simulink model "ME486C_Dyno_DAQ_Quality_Development"  (R2025a)
settings: Solver=FixedStepAuto  StartTime=0.0  StopTime=inf  FixedStep=0.02  RelTol=1e-3  EnableMultiTasking=on
libraries: arduinolib x24, simulink x19
(part 1 of 2)
settings Model: SILPILModeSetting=veronly  ExtModeTrigDuration=2  Creator=YHQ  LastModifiedBy=YHQ
settings OptimizationCC: EnhancedBackFolding=on  PassReuseOutputArgsAs=Individual arguments  ZeroExternalMemoryAtStartup=off  ZeroInternalMemoryAtStartup=off  MaxStackSize=64  OptimizeBlockOrder=speed  DifferentSizesBufferReuse=on  OptimizationCustomize=off  EfficientTunableParamExpr=on
settings DebuggingCC: ParameterTunabilityLossMsg=error
settings HardwareCC: ProdBitPerPointer=32.0  ProdBitPerSizeT=32.0  ProdBitPerPtrDiffT=32.0  ProdLargestAtomicInteger=Long  ProdLargestAtomicFloat=Double  ProdWordSize=32.0  ProdLongLongMode=on  ProdHWDeviceType=ARM Compatible->ARM Cortex  UseEmbeddedCoderFeatures=off  UseSimulinkCoderFeatures=off
settings SFSimCC: MATLABDynamicMemAlloc=off
settings RTWCC: SystemTargetFile=ert.tlc  HardwareBoard=Arduino Uno R4 Minima  TemplateMakefile=ert_default_tmf  Toolchain=Arduino ARM M4  BuildConfiguration=Faster Runs  Description=Embedded Coder
settings CodeAppCC: ForceParamTrailComments=on  IgnoreCustomStorageClasses=off  OperatorAnnotations=on  SimulinkDataObjDesc=on  SFDataObjDesc=on  InsertBlockDesc=on
settings ERTTargetCC: ExtModeTransport=3.0  ExtModeAutomaticAllocSize=off  ExtModeStaticAllocSize=8192.0  InlinedParameterPlacement=Hierarchical  SupportContinuousTime=on  SupportNonInlinedSFcns=on  SupportVariableSizeSignals=on

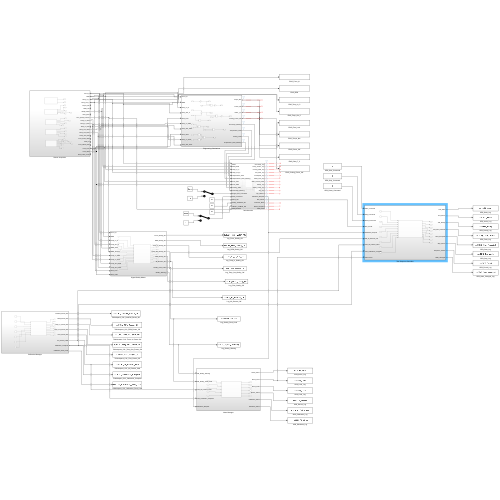
[thumbnail: Simulink's stored preview of the top-level diagram]
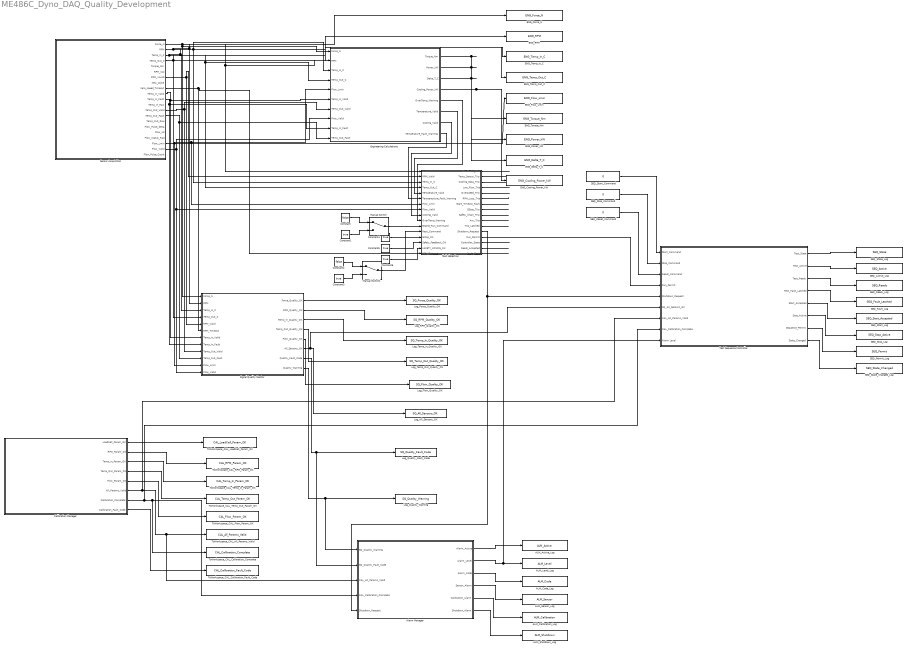
== system ME486C_Dyno_DAQ_Quality_Development ==
  ALM_Active_Log : ToWorkspace  VariableName=ALM_Active  SaveFormat=Timeseries  SampleTime=-1
  ALM_Calibration_Log : ToWorkspace  VariableName=ALM_Calibration  SaveFormat=Timeseries  SampleTime=-1
  ALM_Code_Log : ToWorkspace  VariableName=ALM_Code  SaveFormat=Timeseries  SampleTime=-1
  ALM_Level_Log : ToWorkspace  VariableName=ALM_Level  SaveFormat=Timeseries  SampleTime=-1
  ALM_Sensor_Log : ToWorkspace  VariableName=ALM_Sensor  SaveFormat=Timeseries  SampleTime=-1
  ALM_Shutdown_Log : ToWorkspace  VariableName=ALM_Shutdown  SaveFormat=Timeseries  SampleTime=-1
  Alarm Manager : Subsystem
  Calibration Manager : Subsystem
  Constant : Constant  Value=false  OutDataTypeStr=boolean
  Constant{1,3..6} (5 alike) : Constant  Value=true  OutDataTypeStr=boolean
  Constant2 : Constant  Value=false  OutDataTypeStr=boolean
  ENG_Cooling_Power_kW : ToWorkspace  VariableName=ENG_Cooling_Power_kW  SaveFormat=Timeseries  SampleTime=-1
  ENG_Delta_T_C : ToWorkspace  VariableName=ENG_Delta_T_C  SaveFormat=Timeseries  SampleTime=-1
  ENG_Flow_Lmin : ToWorkspace  VariableName=ENG_Flow_Lmin  SaveFormat=Timeseries  SampleTime=-1
  ENG_Force_N : ToWorkspace  VariableName=ENG_Force_N  SaveFormat=Timeseries  SampleTime=-1
  ENG_Power_kW : ToWorkspace  VariableName=ENG_Power_kW  SaveFormat=Timeseries  SampleTime=-1
  ENG_RPM : ToWorkspace  VariableName=ENG_RPM  SaveFormat=Timeseries  SampleTime=-1
  ENG_Temp_In_C : ToWorkspace  VariableName=ENG_Temp_In_C  SaveFormat=Timeseries  SampleTime=-1
  ENG_Temp_Out_C : ToWorkspace  VariableName=ENG_Temp_Out_C  SaveFormat=Timeseries  SampleTime=-1
  ENG_Torque_Nm : ToWorkspace  VariableName=ENG_Torque_Nm  SaveFormat=Timeseries  SampleTime=-1
  Engineering Calculations : Subsystem
  Log_All_Sensors_OK : ToWorkspace  VariableName=SQ_All_Sensors_OK  SaveFormat=Timeseries  SampleTime=-1
  Log_Flow_Quality_OK : ToWorkspace  VariableName=SQ_Flow_Quality_OK  SaveFormat=Timeseries  SampleTime=-1
  Log_Force_Quality_OK : ToWorkspace  VariableName=SQ_Force_Quality_OK  SaveFormat=Timeseries  SampleTime=-1
  Log_Quality_Fault_Code : ToWorkspace  VariableName=SQ_Quality_Fault_Code  SaveFormat=Timeseries  SampleTime=-1
  Log_Quality_Warning : ToWorkspace  VariableName=SQ_Quality_Warning  SaveFormat=Timeseries  SampleTime=-1
  Log_RPM_Quality_OK : ToWorkspace  VariableName=SQ_RPM_Quality_OK  SaveFormat=Timeseries  SampleTime=-1
  Log_Temp_In_Quality_OK : ToWorkspace  VariableName=SQ_Temp_In_Quality_OK  SaveFormat=Timeseries  SampleTime=-1
  Log_Temp_Out_Quality_OK : ToWorkspace  VariableName=SQ_Temp_Out_Quality_OK  SaveFormat=Timeseries  SampleTime=-1
  Manual Switch : ManualSwitch
  Manual Switch1 : ManualSwitch
  SEQ_Active_Log : ToWorkspace  VariableName=SEQ_Active  SaveFormat=Timeseries  SampleTime=-1
  SEQ_Fault_Log : ToWorkspace  VariableName=SEQ_Fault_Latched  SaveFormat=Timeseries  SampleTime=-1
  SEQ_Permit_Log : ToWorkspace  VariableName=SEQ_Permit  SaveFormat=Timeseries  SampleTime=-1
  SEQ_Ready_Log : ToWorkspace  VariableName=SEQ_Ready  SaveFormat=Timeseries  SampleTime=-1
  SEQ_Reset_Command : Constant  Value=0  OutDataTypeStr=boolean  SampleTime=0.02
  SEQ_Start_Command : Constant  Value=0  OutDataTypeStr=boolean  SampleTime=0.02
  SEQ_Start_Log : ToWorkspace  VariableName=SEQ_Start_Accepted  SaveFormat=Timeseries  SampleTime=-1
  SEQ_State_Changed_Log : ToWorkspace  VariableName=SEQ_State_Changed  SaveFormat=Timeseries  SampleTime=-1
  SEQ_State_Log : ToWorkspace  VariableName=SEQ_State  SaveFormat=Timeseries  SampleTime=-1
  SEQ_Stop_Command : Constant  Value=0  OutDataTypeStr=boolean  SampleTime=0.02
  SEQ_Stop_Log : ToWorkspace  VariableName=SEQ_Stop_Active  SaveFormat=Timeseries  SampleTime=-1
  Sensor Acquisition : Subsystem
  Signal Quality Mentor : Subsystem
  Test Sequence Controller : Subsystem
  ToWorkspace_CAL_All_Params_Valid : ToWorkspace  VariableName=CAL_All_Params_Valid  SaveFormat=Timeseries  SampleTime=-1
  ToWorkspace_CAL_Calibration_Complete : ToWorkspace  VariableName=CAL_Calibration_Complete  SaveFormat=Timeseries  SampleTime=-1
  ToWorkspace_CAL_Calibration_Fault_Code : ToWorkspace  VariableName=CAL_Calibration_Fault_Code  SaveFormat=Timeseries  SampleTime=-1
  ToWorkspace_CAL_Flow_Param_OK : ToWorkspace  VariableName=CAL_Flow_Param_OK  SaveFormat=Timeseries  SampleTime=-1
  ToWorkspace_CAL_LoadCell_Param_OK : ToWorkspace  VariableName=CAL_LoadCell_Param_OK  SaveFormat=Timeseries  SampleTime=-1
  ToWorkspace_CAL_RPM_Param_OK : ToWorkspace  VariableName=CAL_RPM_Param_OK  SaveFormat=Timeseries  SampleTime=-1
  ToWorkspace_CAL_Temp_In_Param_OK : ToWorkspace  VariableName=CAL_Temp_In_Param_OK  SaveFormat=Timeseries  SampleTime=-1
  ToWorkspace_CAL_Temp_Out_Param_OK : ToWorkspace  VariableName=CAL_Temp_Out_Param_OK  SaveFormat=Timeseries  SampleTime=-1
  fault detection : Subsystem
  wires:
  Sensor Acquisition/1(Force_N) -> Engineering Calculations/1(Force_N), Signal Quality Mentor/1(Force_N), ENG_Force_N/1
  Sensor Acquisition/2(RPM) -> fault detection/1(RPM), Engineering Calculations/2(RPM), Signal Quality Mentor/2(RPM), ENG_RPM/1
  Sensor Acquisition/3(Temp_In_C) -> fault detection/3(Temp_In_C), Engineering Calculations/3(Temp_In_C), Signal Quality Mentor/3(Temp_In_C), ENG_Temp_In_C/1
  Sensor Acquisition/4(Temp_Out_C) -> ENG_Temp_Out_C/1, fault detection/4(Temp_Out_C), Engineering Calculations/4(Temp_Out_C), Signal Quality Mentor/4(Temp_Out_C)
  Sensor Acquisition/19(Flow_Lmin) -> ENG_Flow_Lmin/1, Engineering Calculations/5(Flow_Lmin), fault detection/7(Flow_Lmin), Signal Quality Mentor/11(Flow_Lmin)
  Sensor Acquisition/10(Temp_In_Valid) -> Engineering Calculations/6(Temp_In_Valid), Signal Quality Mentor/7(Temp_In_Valid)
  Sensor Acquisition/13(Temp_Out_Valid) -> Engineering Calculations/7(Temp_Out_Valid), Signal Quality Mentor/9(Temp_Out_Valid)
  Sensor Acquisition/11(Temp_In_Fault) -> Engineering Calculations/9(Temp_In_Fault), Signal Quality Mentor/8(Temp_In_Fault)
  Sensor Acquisition/14(Temp_Out_Fault) -> Engineering Calculations/10(Temp_Out_Fault), Signal Quality Mentor/10(Temp_Out_Fault)
  Engineering Calculations/6(Temperature_Valid) -> fault detection/5(Temperature_Valid)
  Engineering Calculations/7(Cooling_Valid) -> fault detection/9(Cooling_Valid)
  Engineering Calculations/8(Temperature_Fault_Warning) -> fault detection/6(Temperasture_Fault_Warning)
  Sensor Acquisition/7(RPM_VALID) -> fault detection/2(RPM_Valid), Signal Quality Mentor/5(RPM_Valid)
  Sensor Acquisition/9(zero_speed_Timeout) -> Signal Quality Mentor/6(RPM_Timeout), fault detection/16(RPM_Timeout)
  Constant/1 -> Manual Switch/1
  Constant1/1 -> Manual Switch/2
  Manual Switch/1 -> fault detection/11(Engine_Run_Command)
  Constant3/1 -> Manual Switch1/2
  Constant2/1 -> Manual Switch1/1
  Manual Switch1/1 -> fault detection/12(Rest_Command)
  Constant4/1 -> fault detection/13(Estop_OK)
  Constant5/1 -> fault detection/14(Safety_Feedback_OK)
  Constant6/1 -> fault detection/15(sAFETY_cONFIG_OK)
  Engineering Calculations/5(OverTemp_Warning) -> fault detection/10(OverTemp_Warning)
  fault detection/1(OverTemp_Trip) -> ?
  fault detection/2(Temp_Sensor_Trip) -> ?
  fault detection/3(Cooling_Data_Trip) -> ?
  fault detection/4(Low_Flow_Trip) -> ?
  fault detection/5(Overspeed_Trip) -> ?
  fault detection/6(RPM_Loss_Trip) -> ?
  fault detection/7(Start_Timeout_Fault) -> ?
  fault detection/8(EStop_Trip) -> ?
  fault detection/9(Safety_Chain_Trip) -> ?
  fault detection/10(Any_Trip) -> ?
  fault detection/11(Trip_Latched) -> ?
  fault detection/12(Shutdown_Request) -> Alarm Manager/5(Shutdown_Request), Test Sequence Controller/5(Shutdown_Request)
  fault detection/13(Run_Permit) -> Test Sequence Controller/4(Run_Permit)
  fault detection/14(Controller_State) -> ?
  fault detection/15(Reset_Accepted) -> ?
  fault detection/16(Fault_Code) -> ?
  Engineering Calculations/1(Torque_Nm) -> ENG_Torque_Nm/1
  Engineering Calculations/2(Power_kW) -> ENG_Power_kW/1
  Engineering Calculations/3(Delta_T_C) -> ENG_Delta_T_C/1
  Engineering Calculations/4(Cooling_Power_kW) -> ENG_Cooling_Power_kW/1
  Sensor Acquisition/20(Flow_Valid) -> Engineering Calculations/8(Flow_Valid), Signal Quality Mentor/12(Flow_Valid), fault detection/8(Flow_Valid)
  Signal Quality Mentor/1(Force_Quality_OK) -> Log_Force_Quality_OK/1
  Signal Quality Mentor/2(RPM_Quality_OK) -> Log_RPM_Quality_OK/1
  Signal Quality Mentor/3(Temp_In_Quality_OK) -> Log_Temp_In_Quality_OK/1
  Signal Quality Mentor/4(Temp_Out_Quality_OK) -> Log_Temp_Out_Quality_OK/1
  Signal Quality Mentor/5(Flow_Quality_OK) -> Log_Flow_Quality_OK/1
  Signal Quality Mentor/6(All_Sensors_OK) -> Test Sequence Controller/6(SQ_All_Sensors_OK), Log_All_Sensors_OK/1
  Signal Quality Mentor/7(Quality_Fault_Code) -> Alarm Manager/2(SQ_Quality_Fault_Code), Log_Quality_Fault_Code/1
  Signal Quality Mentor/8(Quality_Warning) -> Alarm Manager/1(SQ_Quality_Warning), Log_Quality_Warning/1
  Calibration Manager/1(LoadCell_Param_OK) -> ToWorkspace_CAL_LoadCell_Param_OK/1
  Calibration Manager/2(RPM_Param_OK) -> ToWorkspace_CAL_RPM_Param_OK/1
  Calibration Manager/3(Temp_In_Param_OK) -> ToWorkspace_CAL_Temp_In_Param_OK/1
  Calibration Manager/4(Temp_Out_Param_OK) -> ToWorkspace_CAL_Temp_Out_Param_OK/1
  Calibration Manager/5(Flow_Param_OK) -> ToWorkspace_CAL_Flow_Param_OK/1
  Calibration Manager/6(All_Params_Valid) -> Test Sequence Controller/7(CAL_All_Params_Valid), Alarm Manager/3(CAL_All_Params_Valid), ToWorkspace_CAL_All_Params_Valid/1
  Calibration Manager/7(Calibration_Complete) -> Alarm Manager/4(CAL_Calibration_Complete), ToWorkspace_CAL_Calibration_Complete/1, Test Sequence Controller/8(CAL_Calibration_Complete)
  Calibration Manager/8(Calibration_Fault_Code) -> ToWorkspace_CAL_Calibration_Fault_Code/1
  Alarm Manager/1(Alarm_Active) -> ALM_Active_Log/1
  Alarm Manager/2(Alarm_Level) -> Test Sequence Controller/9(Alarm Level), ALM_Level_Log/1
  Alarm Manager/3(Alarm_Code) -> ALM_Code_Log/1
  Alarm Manager/4(Sensor_Alarm) -> ALM_Sensor_Log/1
  Alarm Manager/5(Calibration_Alarm) -> ALM_Calibration_Log/1
  Alarm Manager/6(Shutdown_Alarm) -> ALM_Shutdown_Log/1
  SEQ_Start_Command/1 -> Test Sequence Controller/1(Start_Command)
  SEQ_Stop_Command/1 -> Test Sequence Controller/2(Stop_Command)
  SEQ_Reset_Command/1 -> Test Sequence Controller/3(Reset_Command)
  Test Sequence Controller/1(Test_State) -> SEQ_State_Log/1
  Test Sequence Controller/2(Test_Active) -> SEQ_Active_Log/1
  Test Sequence Controller/3(Test_Ready) -> SEQ_Ready_Log/1
  Test Sequence Controller/4(Test_Fault_Latched) -> SEQ_Fault_Log/1
  Test Sequence Controller/5(Start_Accepted) -> SEQ_Start_Log/1
  Test Sequence Controller/6(Stop_Active) -> SEQ_Stop_Log/1
  Test Sequence Controller/7(Sequence_Permit) -> SEQ_Permit_Log/1
  Test Sequence Controller/8(State_Changed) -> SEQ_State_Changed_Log/1

== system ME486C_Dyno_DAQ_Quality_Development/Alarm Manager ==
  SQ_Quality_Warning : Inport
  SQ_Quality_Fault_Code : Inport  Port=2
  CAL_All_Params_Valid : Inport  Port=3
  CAL_Calibration_Complete : Inport  Port=4
  Shutdown_Request : Inport  Port=5
  Alarm_Logic_Core : MATLAB Function  TreatAsAtomicUnit=on
  Alarm_Active : Outport
  Alarm_Level : Outport  Port=2
  Alarm_Code : Outport  Port=3
  Sensor_Alarm : Outport  Port=4
  Calibration_Alarm : Outport  Port=5
  Shutdown_Alarm : Outport  Port=6
  wires:
  Shutdown_Request/1 -> Alarm_Logic_Core/5(Shutdown_Request)
  CAL_Calibration_Complete/1 -> Alarm_Logic_Core/4(CAL_Calibration_Complete)
  CAL_All_Params_Valid/1 -> Alarm_Logic_Core/3(CAL_All_Params_Valid)
  SQ_Quality_Fault_Code/1 -> Alarm_Logic_Core/2(SQ_Quality_Fault_Code)
  SQ_Quality_Warning/1 -> Alarm_Logic_Core/1(SQ_Quality_Warning)
  Alarm_Logic_Core/1(Alarm_Active) -> Alarm_Active/1
  Alarm_Logic_Core/2(Alarm_Level) -> Alarm_Level/1
  Alarm_Logic_Core/3(Alarm_Code) -> Alarm_Code/1
  Alarm_Logic_Core/4(Sensor_Alarm) -> Sensor_Alarm/1
  Alarm_Logic_Core/5(Calibration_Alarm) -> Calibration_Alarm/1
  Alarm_Logic_Core/6(Shutdown_Alarm) -> Shutdown_Alarm/1

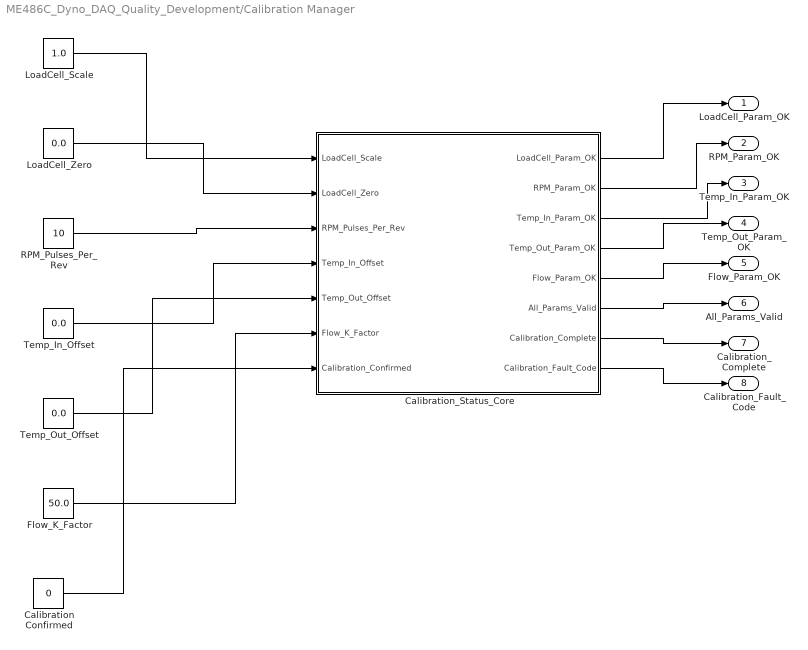
== system ME486C_Dyno_DAQ_Quality_Development/Calibration Manager ==
  Calibration Confirmed : Constant  Value=0  OutDataTypeStr=boolean
  Calibration_Status_Core : MATLAB Function  TreatAsAtomicUnit=on
  Flow_K_Factor : Constant  Value=50.0
  LoadCell_Scale : Constant  Value=1.0
  LoadCell_Zero : Constant  Value=0.0
  RPM_Pulses_Per_Rev : Constant  Value=10
  Temp_In_Offset : Constant  Value=0.0
  Temp_Out_Offset : Constant  Value=0.0
  LoadCell_Param_OK : Outport
  RPM_Param_OK : Outport  Port=2
  Temp_In_Param_OK : Outport  Port=3
  Temp_Out_Param_OK : Outport  Port=4
  Flow_Param_OK : Outport  Port=5
  All_Params_Valid : Outport  Port=6
  Calibration_Complete : Outport  Port=7
  Calibration_Fault_Code : Outport  Port=8
  wires:
  LoadCell_Scale/1 -> Calibration_Status_Core/1(LoadCell_Scale)
  LoadCell_Zero/1 -> Calibration_Status_Core/2(LoadCell_Zero)
  RPM_Pulses_Per_Rev/1 -> Calibration_Status_Core/3(RPM_Pulses_Per_Rev)
  Temp_In_Offset/1 -> Calibration_Status_Core/4(Temp_In_Offset)
  Temp_Out_Offset/1 -> Calibration_Status_Core/5(Temp_Out_Offset)
  Flow_K_Factor/1 -> Calibration_Status_Core/6(Flow_K_Factor)
  Calibration_Status_Core/1(LoadCell_Param_OK) -> LoadCell_Param_OK/1
  Calibration_Status_Core/2(RPM_Param_OK) -> RPM_Param_OK/1
  Calibration_Status_Core/3(Temp_In_Param_OK) -> Temp_In_Param_OK/1
  Calibration_Status_Core/4(Temp_Out_Param_OK) -> Temp_Out_Param_OK/1
  Calibration_Status_Core/5(Flow_Param_OK) -> Flow_Param_OK/1
  Calibration_Status_Core/6(All_Params_Valid) -> All_Params_Valid/1
  Calibration_Status_Core/7(Calibration_Complete) -> Calibration_Complete/1
  Calibration_Status_Core/8(Calibration_Fault_Code) -> Calibration_Fault_Code/1
  Calibration Confirmed/1 -> Calibration_Status_Core/7(Calibration_Confirmed)

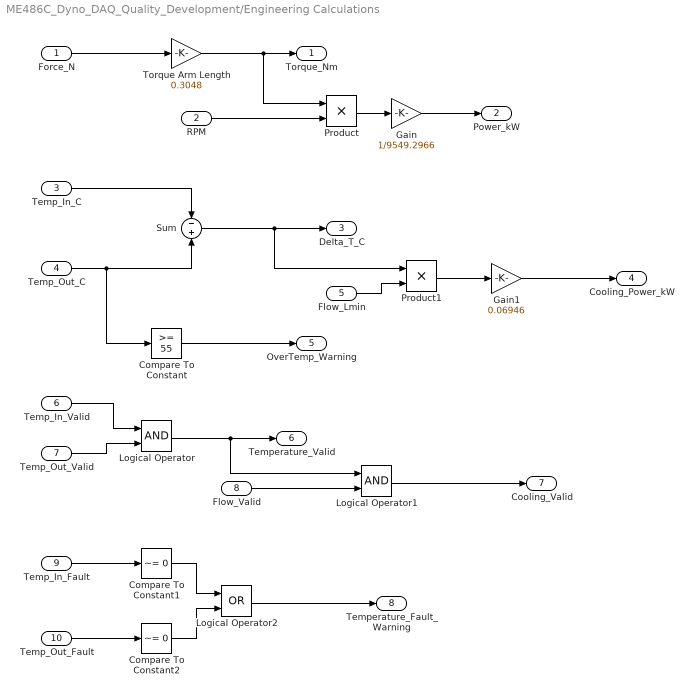
== system ME486C_Dyno_DAQ_Quality_Development/Engineering Calculations ==
  Force_N : Inport
  RPM : Inport  Port=2
  Temp_In_C : Inport  Port=3
  Temp_Out_C : Inport  Port=4
  Flow_Lmin : Inport  Port=5
  Temp_In_Valid : Inport  Port=6
  Temp_Out_Valid : Inport  Port=7
  Flow_Valid : Inport  Port=8
  Temp_In_Fault : Inport  Port=9
  Temp_Out_Fault : Inport  Port=10
  Compare To Constant : simulink/Logic and Bit Operations/Compare To Constant  relop=>=  const=55  OutDataTypeStr=boolean
  Compare To Constant1 : simulink/Logic and Bit Operations/Compare To Constant  relop=~=  const=0  OutDataTypeStr=boolean
  Compare To Constant2 : simulink/Logic and Bit Operations/Compare To Constant  relop=~=  const=0  OutDataTypeStr=boolean
  Gain : Gain  Gain=1/9549.2966
  Gain1 : Gain  Gain=0.06946
  Logical Operator : Logic  AllPortsSameDT=off  OutDataTypeStr=boolean
  Logical Operator1 : Logic  AllPortsSameDT=off  OutDataTypeStr=boolean
  Logical Operator2 : Logic  Operator=OR  AllPortsSameDT=off  OutDataTypeStr=boolean
  Product : Product
  Product1 : Product
  Sum : Sum  Inputs=-+
  Torque Arm Length : Gain  Gain=0.3048
  Torque_Nm : Outport
  Power_kW : Outport  Port=2
  Delta_T_C : Outport  Port=3
  Cooling_Power_kW : Outport  Port=4
  OverTemp_Warning : Outport  Port=5
  Temperature_Valid : Outport  Port=6
  Cooling_Valid : Outport  Port=7
  Temperature_Fault_Warning : Outport  Port=8
  wires:
  Force_N/1 -> Torque Arm Length/1
  Torque Arm Length/1 -> Product/1, Torque_Nm/1
  RPM/1 -> Product/2
  Product/1 -> Gain/1
  Gain/1 -> Power_kW/1
  Temp_In_C/1 -> Sum/1
  Temp_Out_C/1 -> Compare To Constant/1, Sum/2
  Sum/1 -> Product1/1, Delta_T_C/1
  Flow_Lmin/1 -> Product1/2
  Product1/1 -> Gain1/1
  Gain1/1 -> Cooling_Power_kW/1
  Compare To Constant/1 -> OverTemp_Warning/1
  Temp_In_Valid/1 -> Logical Operator/1
  Temp_Out_Valid/1 -> Logical Operator/2
  Logical Operator/1 -> Logical Operator1/1, Temperature_Valid/1
  Flow_Valid/1 -> Logical Operator1/2
  Logical Operator1/1 -> Cooling_Valid/1
  Temp_In_Fault/1 -> Compare To Constant1/1
  Temp_Out_Fault/1 -> Compare To Constant2/1
  Compare To Constant1/1 -> Logical Operator2/1
  Compare To Constant2/1 -> Logical Operator2/2
  Logical Operator2/1 -> Temperature_Fault_Warning/1

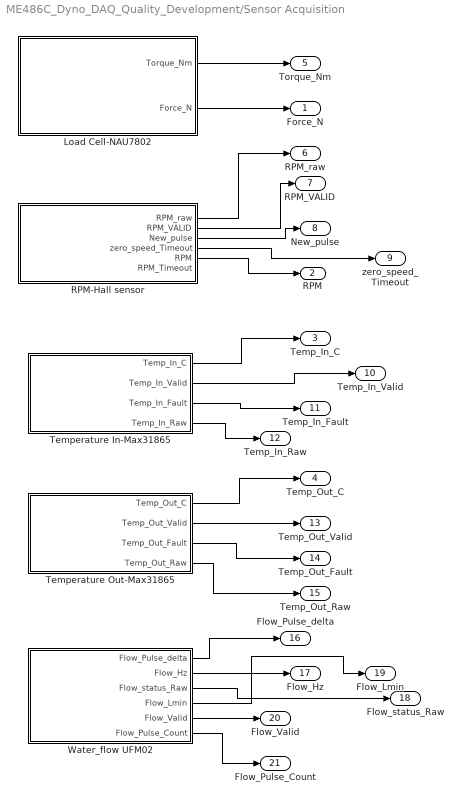
== system ME486C_Dyno_DAQ_Quality_Development/Sensor Acquisition ==
  Load Cell-NAU7802 : Subsystem
  RPM-Hall sensor : Subsystem
  Temperature In-Max31865 : Subsystem
  Temperature Out-Max31865 : Subsystem
  Water_flow UFM02 : Subsystem
  Force_N : Outport
  RPM : Outport  Port=2
  Temp_In_C : Outport  Port=3
  Temp_Out_C : Outport  Port=4
  Torque_Nm : Outport  Port=5
  RPM_raw : Outport  Port=6
  RPM_VALID : Outport  Port=7
  New_pulse : Outport  Port=8
  zero_speed_Timeout : Outport  Port=9
  Temp_In_Valid : Outport  Port=10
  Temp_In_Fault : Outport  Port=11
  Temp_In_Raw : Outport  Port=12
  Temp_Out_Valid : Outport  Port=13
  Temp_Out_Fault : Outport  Port=14
  Temp_Out_Raw : Outport  Port=15
  Flow_Pulse_delta : Outport  Port=16
  Flow_Hz : Outport  Port=17
  Flow_status_Raw : Outport  Port=18
  Flow_Lmin : Outport  Port=19
  Flow_Valid : Outport  Port=20
  Flow_Pulse_Count : Outport  Port=21
  wires:
  Load Cell-NAU7802/2(Force_N) -> Force_N/1
  RPM-Hall sensor/5(RPM) -> RPM/1
  Temperature In-Max31865/1(Temp_In_C) -> Temp_In_C/1
  Temperature Out-Max31865/1(Temp_Out_C) -> Temp_Out_C/1
  Load Cell-NAU7802/1(Torque_Nm) -> Torque_Nm/1
  RPM-Hall sensor/1(RPM_raw) -> RPM_raw/1
  RPM-Hall sensor/2(RPM_VALID) -> RPM_VALID/1
  RPM-Hall sensor/3(New_pulse) -> New_pulse/1
  RPM-Hall sensor/4(zero_speed_Timeout) -> zero_speed_Timeout/1
  Temperature In-Max31865/2(Temp_In_Valid) -> Temp_In_Valid/1
  Temperature In-Max31865/3(Temp_In_Fault) -> Temp_In_Fault/1
  Temperature In-Max31865/4(Temp_In_Raw) -> Temp_In_Raw/1
  Temperature Out-Max31865/2(Temp_Out_Valid) -> Temp_Out_Valid/1
  Temperature Out-Max31865/3(Temp_Out_Fault) -> Temp_Out_Fault/1
  Temperature Out-Max31865/4(Temp_Out_Raw) -> Temp_Out_Raw/1
  Water_flow UFM02/1(Flow_Pulse_delta) -> Flow_Pulse_delta/1
  Water_flow UFM02/2(Flow_Hz) -> Flow_Hz/1
  Water_flow UFM02/3(Flow_status_Raw) -> Flow_status_Raw/1
  Water_flow UFM02/4(Flow_Lmin) -> Flow_Lmin/1
  Water_flow UFM02/5(Flow_Valid) -> Flow_Valid/1
  Water_flow UFM02/6(Flow_Pulse_Count) -> Flow_Pulse_Count/1

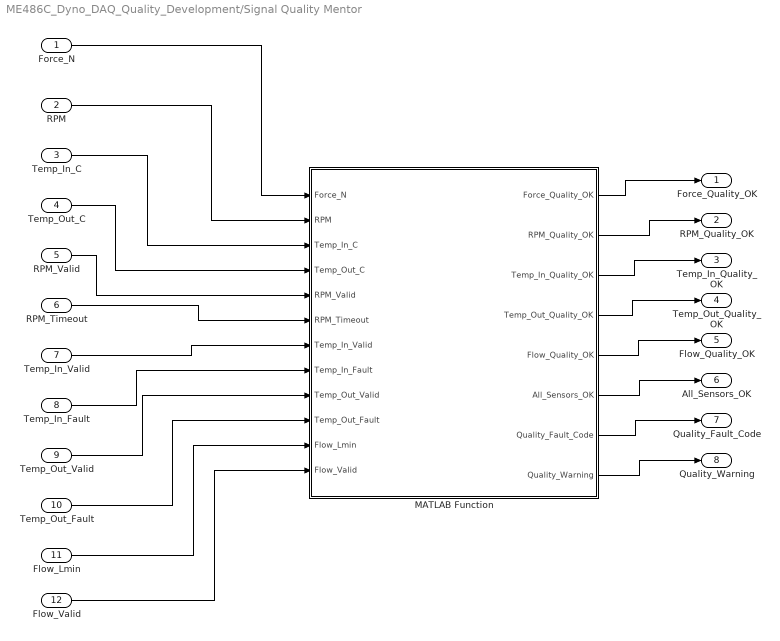
== system ME486C_Dyno_DAQ_Quality_Development/Signal Quality Mentor ==
  Force_N : Inport
  RPM : Inport  Port=2
  Temp_In_C : Inport  Port=3
  Temp_Out_C : Inport  Port=4
  RPM_Valid : Inport  Port=5
  RPM_Timeout : Inport  Port=6
  Temp_In_Valid : Inport  Port=7
  Temp_In_Fault : Inport  Port=8
  Temp_Out_Valid : Inport  Port=9
  Temp_Out_Fault : Inport  Port=10
  Flow_Lmin : Inport  Port=11
  Flow_Valid : Inport  Port=12
  MATLAB Function : MATLAB Function  TreatAsAtomicUnit=on
  Force_Quality_OK : Outport
  RPM_Quality_OK : Outport  Port=2
  Temp_In_Quality_OK : Outport  Port=3
  Temp_Out_Quality_OK : Outport  Port=4
  Flow_Quality_OK : Outport  Port=5
  All_Sensors_OK : Outport  Port=6
  Quality_Fault_Code : Outport  Port=7
  Quality_Warning : Outport  Port=8
  wires:
  Force_N/1 -> MATLAB Function/1(Force_N)
  RPM/1 -> MATLAB Function/2(RPM)
  MATLAB Function/1(Force_Quality_OK) -> Force_Quality_OK/1
  MATLAB Function/2(RPM_Quality_OK) -> RPM_Quality_OK/1
  Temp_In_C/1 -> MATLAB Function/3(Temp_In_C)
  Temp_Out_C/1 -> MATLAB Function/4(Temp_Out_C)
  RPM_Valid/1 -> MATLAB Function/5(RPM_Valid)
  RPM_Timeout/1 -> MATLAB Function/6(RPM_Timeout)
  Temp_In_Valid/1 -> MATLAB Function/7(Temp_In_Valid)
  Temp_In_Fault/1 -> MATLAB Function/8(Temp_In_Fault)
  Temp_Out_Valid/1 -> MATLAB Function/9(Temp_Out_Valid)
  Temp_Out_Fault/1 -> MATLAB Function/10(Temp_Out_Fault)
  Flow_Lmin/1 -> MATLAB Function/11(Flow_Lmin)
  Flow_Valid/1 -> MATLAB Function/12(Flow_Valid)
  MATLAB Function/3(Temp_In_Quality_OK) -> Temp_In_Quality_OK/1
  MATLAB Function/4(Temp_Out_Quality_OK) -> Temp_Out_Quality_OK/1
  MATLAB Function/5(Flow_Quality_OK) -> Flow_Quality_OK/1
  MATLAB Function/6(All_Sensors_OK) -> All_Sensors_OK/1
  MATLAB Function/7(Quality_Fault_Code) -> Quality_Fault_Code/1
  MATLAB Function/8(Quality_Warning) -> Quality_Warning/1

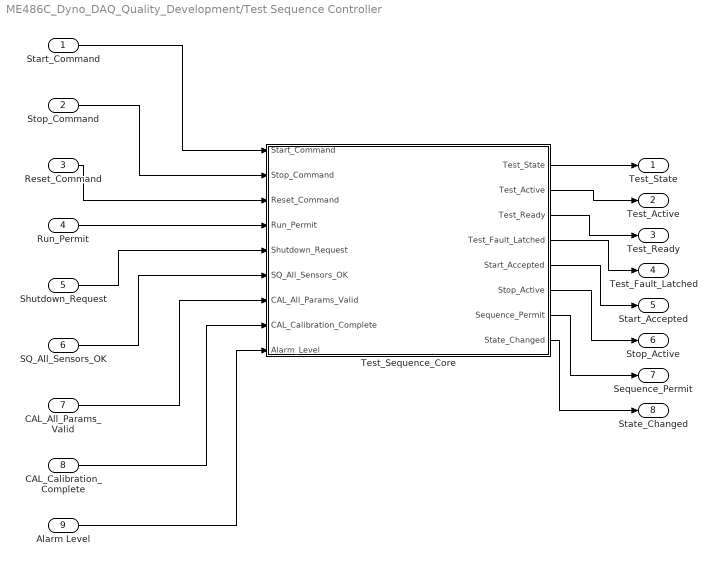
== system ME486C_Dyno_DAQ_Quality_Development/Test Sequence Controller ==
  Start_Command : Inport
  Stop_Command : Inport  Port=2
  Reset_Command : Inport  Port=3
  Run_Permit : Inport  Port=4
  Shutdown_Request : Inport  Port=5
  SQ_All_Sensors_OK : Inport  Port=6
  CAL_All_Params_Valid : Inport  Port=7
  CAL_Calibration_Complete : Inport  Port=8
  Alarm Level : Inport  Port=9
  Test_Sequence_Core : MATLAB Function  TreatAsAtomicUnit=on
  Test_State : Outport
  Test_Active : Outport  Port=2
  Test_Ready : Outport  Port=3
  Test_Fault_Latched : Outport  Port=4
  Start_Accepted : Outport  Port=5
  Stop_Active : Outport  Port=6
  Sequence_Permit : Outport  Port=7
  State_Changed : Outport  Port=8
  wires:
  Start_Command/1 -> Test_Sequence_Core/1(Start_Command)
  Stop_Command/1 -> Test_Sequence_Core/2(Stop_Command)
  Reset_Command/1 -> Test_Sequence_Core/3(Reset_Command)
  Run_Permit/1 -> Test_Sequence_Core/4(Run_Permit)
  Shutdown_Request/1 -> Test_Sequence_Core/5(Shutdown_Request)
  SQ_All_Sensors_OK/1 -> Test_Sequence_Core/6(SQ_All_Sensors_OK)
  CAL_All_Params_Valid/1 -> Test_Sequence_Core/7(CAL_All_Params_Valid)
  CAL_Calibration_Complete/1 -> Test_Sequence_Core/8(CAL_Calibration_Complete)
  Alarm Level/1 -> Test_Sequence_Core/9(Alarm_Level)
  Test_Sequence_Core/1(Test_State) -> Test_State/1
  Test_Sequence_Core/2(Test_Active) -> Test_Active/1
  Test_Sequence_Core/3(Test_Ready) -> Test_Ready/1
  Test_Sequence_Core/4(Test_Fault_Latched) -> Test_Fault_Latched/1
  Test_Sequence_Core/5(Start_Accepted) -> Start_Accepted/1
  Test_Sequence_Core/6(Stop_Active) -> Stop_Active/1
  Test_Sequence_Core/7(Sequence_Permit) -> Sequence_Permit/1
  Test_Sequence_Core/8(State_Changed) -> State_Changed/1

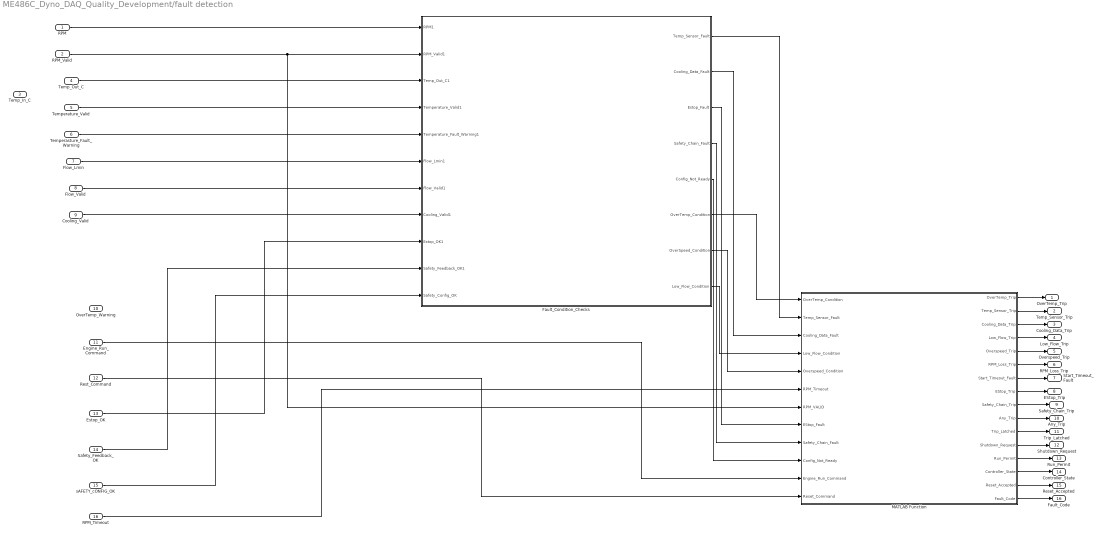
== system ME486C_Dyno_DAQ_Quality_Development/fault detection ==
  RPM : Inport
  RPM_Valid : Inport  Port=2
  Temp_In_C : Inport  Port=3
  Temp_Out_C : Inport  Port=4
  Temperature_Valid : Inport  Port=5
  Temperasture_Fault_Warning : Inport  Port=6
  Flow_Lmin : Inport  Port=7
  Flow_Valid : Inport  Port=8
  Cooling_Valid : Inport  Port=9
  OverTemp_Warning : Inport  Port=10
  Engine_Run_Command : Inport  Port=11
  Rest_Command : Inport  Port=12
  Estop_OK : Inport  Port=13
  Safety_Feedback_OK : Inport  Port=14
  sAFETY_cONFIG_OK : Inport  Port=15
  RPM_Timeout : Inport  Port=16
  Fault_Condition_Checks : Subsystem
  MATLAB Function : MATLAB Function  TreatAsAtomicUnit=on
  OverTemp_Trip : Outport
  Temp_Sensor_Trip : Outport  Port=2
  Cooling_Data_Trip : Outport  Port=3
  Low_Flow_Trip : Outport  Port=4
  Overspeed_Trip : Outport  Port=5
  RPM_Loss_Trip : Outport  Port=6
  Start_Timeout_Fault : Outport  Port=7
  EStop_Trip : Outport  Port=8
  Safety_Chain_Trip : Outport  Port=9
  Any_Trip : Outport  Port=10
  Trip_Latched : Outport  Port=11
  Shutdown_Request : Outport  Port=12
  Run_Permit : Outport  Port=13
  Controller_State : Outport  Port=14
  Reset_Accepted : Outport  Port=15
  Fault_Code : Outport  Port=16
  wires:
  RPM/1 -> Fault_Condition_Checks/1(RPM1)
  RPM_Valid/1 -> MATLAB Function/7(RPM_VALID), Fault_Condition_Checks/2(RPM_Valid1)
  Temp_Out_C/1 -> Fault_Condition_Checks/3(Temp_Out_C1)
  Temperature_Valid/1 -> Fault_Condition_Checks/4(Temperature_Valid1)
  Temperasture_Fault_Warning/1 -> Fault_Condition_Checks/5(Temperature_Fault_Warning1)
  Flow_Lmin/1 -> Fault_Condition_Checks/6(Flow_Lmin1)
  Flow_Valid/1 -> Fault_Condition_Checks/7(Flow_Valid1)
  Cooling_Valid/1 -> Fault_Condition_Checks/8(Cooling_Valid1)
  Estop_OK/1 -> Fault_Condition_Checks/9(Estop_OK1)
  Safety_Feedback_OK/1 -> Fault_Condition_Checks/10(Safety_Feedback_OK1)
  sAFETY_cONFIG_OK/1 -> Fault_Condition_Checks/11(Safety_Config_OK)
  RPM_Timeout/1 -> MATLAB Function/6(RPM_Timeout)
  Engine_Run_Command/1 -> MATLAB Function/11(Engine_Run_Command)
  Rest_Command/1 -> MATLAB Function/12(Reset_Command)
  Fault_Condition_Checks/6(OverTemp_Condition) -> MATLAB Function/1(OverTemp_Condition)
  Fault_Condition_Checks/1(Temp_Sensor_Fault) -> MATLAB Function/2(Temp_Sensor_Fault)
  Fault_Condition_Checks/2(Cooling_Data_Fault) -> MATLAB Function/3(Cooling_Data_Fault)
  Fault_Condition_Checks/3(Estop_Fault) -> MATLAB Function/8(EStop_Fault)
  Fault_Condition_Checks/4(Safety_Chain_Fault) -> MATLAB Function/9(Safety_Chain_Fault)
  Fault_Condition_Checks/5(Config_Not_Ready) -> MATLAB Function/10(Config_Not_Ready)
  Fault_Condition_Checks/8(Low_Flow_Condition) -> MATLAB Function/4(Low_Flow_Condition)
  Fault_Condition_Checks/7(OverSpeed_Condition) -> MATLAB Function/5(Overspeed_Condition)
  MATLAB Function/1(OverTemp_Trip) -> OverTemp_Trip/1
  MATLAB Function/2(Temp_Sensor_Trip) -> Temp_Sensor_Trip/1
  MATLAB Function/3(Cooling_Data_Trip) -> Cooling_Data_Trip/1
  MATLAB Function/4(Low_Flow_Trip) -> Low_Flow_Trip/1
  MATLAB Function/5(Overspeed_Trip) -> Overspeed_Trip/1
  MATLAB Function/6(RPM_Loss_Trip) -> RPM_Loss_Trip/1
  MATLAB Function/7(Start_Timeout_Fault) -> Start_Timeout_Fault/1
  MATLAB Function/8(EStop_Trip) -> EStop_Trip/1
  MATLAB Function/9(Safety_Chain_Trip) -> Safety_Chain_Trip/1
  MATLAB Function/10(Any_Trip) -> Any_Trip/1
  MATLAB Function/11(Trip_Latched) -> Trip_Latched/1
  MATLAB Function/12(Shutdown_Request) -> Shutdown_Request/1
  MATLAB Function/13(Run_Permit) -> Run_Permit/1
  MATLAB Function/14(Controller_State) -> Controller_State/1
  MATLAB Function/15(Reset_Accepted) -> Reset_Accepted/1
  MATLAB Function/16(Fault_Code) -> Fault_Code/1

== system ME486C_Dyno_DAQ_Quality_Development/Sensor Acquisition/Load Cell-NAU7802 ==
  ADC Data read : Subsystem  TreatAsAtomicUnit=on
  Logical Operator : Logic  AllPortsSameDT=off  OutDataTypeStr=boolean
  NAU7802 Initialization : Subsystem
  Torque Arm length : Gain  Gain=0.3048
  Torque_Nm : Outport
  Force_N : Outport  Port=2
  wires:
  NAU7802 Initialization/2(CR_Status) -> Logical Operator/1
  NAU7802 Initialization/6(Calibration done) -> Logical Operator/2
  Logical Operator/1 -> ADC Data read/Enable
  Torque Arm length/1 -> Torque_Nm/1
  ADC Data read/5(Force_N) -> Force_N/1, Torque Arm length/1

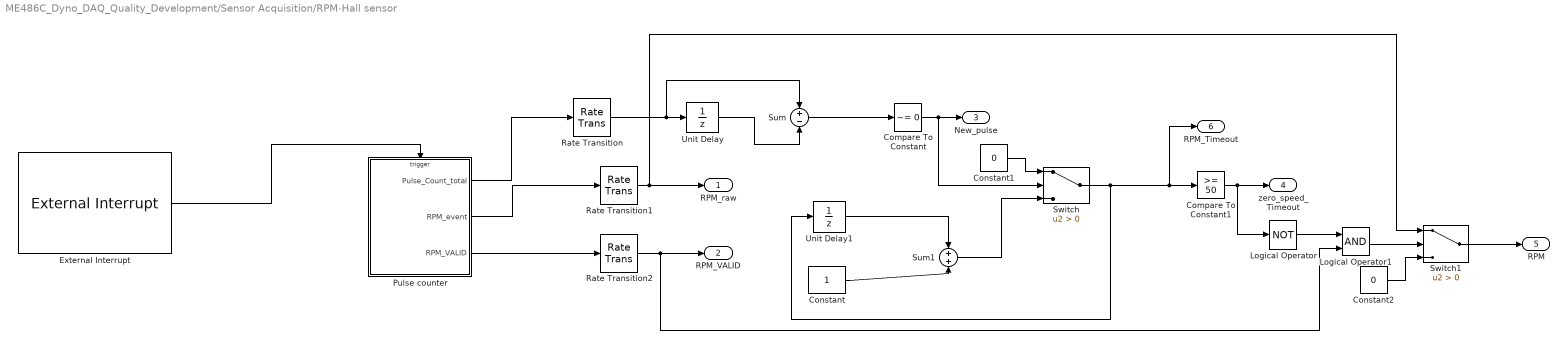
== system ME486C_Dyno_DAQ_Quality_Development/Sensor Acquisition/RPM-Hall sensor ==
  Compare To Constant : simulink/Logic and Bit Operations/Compare To Constant  relop=~=  const=0  OutDataTypeStr=boolean
  Compare To Constant1 : simulink/Logic and Bit Operations/Compare To Constant  relop=>=  const=50  OutDataTypeStr=boolean
  Constant : Constant  OutDataTypeStr=uint16
  Constant1 : Constant  Value=0  OutDataTypeStr=uint16
  Constant2 : Constant  Value=0  OutDataTypeStr=uint16
  External Interrupt : arduinolib/External Interrupt  Pin=2  PullUp=off  Mode=RISING  InterruptSimulationInput=off
  Logical Operator : Logic  Operator=NOT  AllPortsSameDT=off  OutDataTypeStr=boolean
  Logical Operator1 : Logic  AllPortsSameDT=off  OutDataTypeStr=boolean
  Pulse counter : Subsystem  TreatAsAtomicUnit=on
  Rate Transition : RateTransition  Deterministic=off
  Rate Transition1 : RateTransition  Deterministic=off
  Rate Transition2 : RateTransition  Deterministic=off
  Sum : Sum  Inputs=+-
  Sum1 : Sum
  Switch : Switch  Criteria=u2 > Threshold  SaturateOnIntegerOverflow=off  InputSameDT=off
  Switch1 : Switch  Criteria=u2 > Threshold  SaturateOnIntegerOverflow=off  InputSameDT=off
  Unit Delay : UnitDelay  SampleTime=0.02  HasFrameUpgradeWarning=on
  Unit Delay1 : UnitDelay  SampleTime=0.02  HasFrameUpgradeWarning=on
  RPM_raw : Outport
  RPM_VALID : Outport  Port=2
  New_pulse : Outport  Port=3
  zero_speed_Timeout : Outport  Port=4
  RPM : Outport  Port=5
  RPM_Timeout : Outport  Port=6
  wires:
  Pulse counter/2(RPM_event) -> Rate Transition1/1
  Pulse counter/3(RPM_VALID) -> Rate Transition2/1
  Rate Transition1/1 -> RPM_raw/1, Switch1/1
  Rate Transition2/1 -> Logical Operator1/2, RPM_VALID/1
  Pulse counter/1(Pulse_Count_total) -> Rate Transition/1
  Rate Transition/1 -> Sum/1, Unit Delay/1
  Sum/1 -> Compare To Constant/1
  Compare To Constant/1 -> Switch/2, New_pulse/1
  Unit Delay/1 -> Sum/2
  Unit Delay1/1 -> Sum1/1
  Constant/1 -> Sum1/2
  Sum1/1 -> Switch/3
  Constant1/1 -> Switch/1
  Switch/1 -> RPM_Timeout/1, Compare To Constant1/1, Unit Delay1/1
  Compare To Constant1/1 -> Logical Operator/1, zero_speed_Timeout/1
  Logical Operator/1 -> Logical Operator1/1
  Logical Operator1/1 -> Switch1/2
  Constant2/1 -> Switch1/3
  Switch1/1 -> RPM/1
  External Interrupt/1 -> Pulse counter/Trigger

== system ME486C_Dyno_DAQ_Quality_Development/Sensor Acquisition/Temperature In-Max31865 ==
  Fault_Read_Command : Constant  Value=uint8([7 0])
  MAX31865_Temperature Conversion : MATLAB Function  TreatAsAtomicUnit=on
  MAX31865_config : Constant  Value=uint8([128,208])  OutDataTypeStr=uint8
  RTD_Read_command : Constant  Value=uint8([1 0 0])  OutDataTypeStr=uint8
  SPI Read_Fault_In : arduinolib/SPI WriteRead  SPIModule=0  slaveSelectPin_=9  blockPlatform=ARDUINO
  SPI Read_RTD_In : arduinolib/SPI WriteRead  SPIModule=0  slaveSelectPin_=9  blockPlatform=ARDUINO
  SPI_Config_In : arduinolib/SPI WriteRead  SPIModule=0  slaveSelectPin_=9  blockPlatform=ARDUINO
  Temp_In_C : Outport
  Temp_In_Valid : Outport  Port=2
  Temp_In_Fault : Outport  Port=3
  Temp_In_Raw : Outport  Port=4
  wires:
  MAX31865_config/1 -> SPI_Config_In/1
  RTD_Read_command/1 -> SPI Read_RTD_In/1
  Fault_Read_Command/1 -> SPI Read_Fault_In/1
  SPI Read_RTD_In/1 -> MAX31865_Temperature Conversion/1(rtdBytes)
  SPI Read_Fault_In/1 -> MAX31865_Temperature Conversion/2(faultBytes)
  MAX31865_Temperature Conversion/1(Temp_In_C) -> Temp_In_C/1
  MAX31865_Temperature Conversion/2(Temp_In_Valid) -> Temp_In_Valid/1
  MAX31865_Temperature Conversion/3(Temp_In_Fault) -> Temp_In_Fault/1
  MAX31865_Temperature Conversion/4(Temp_In_Raw) -> Temp_In_Raw/1

== system ME486C_Dyno_DAQ_Quality_Development/Sensor Acquisition/Temperature Out-Max31865 ==
  Fault_Read_Command : Constant  Value=uint8([7 0])
  MAX31865_Temperature Conversion : MATLAB Function  TreatAsAtomicUnit=on
  MAX31865_config : Constant  Value=uint8([128,208])  OutDataTypeStr=uint8
  RTD_Read_command : Constant  Value=uint8([1 0 0])  OutDataTypeStr=uint8
  SPI Read_Fault_out : arduinolib/SPI WriteRead  SPIModule=0  slaveSelectPin_=10  blockPlatform=ARDUINO
  SPI Read_RTD_out : arduinolib/SPI WriteRead  SPIModule=0  slaveSelectPin_=10  blockPlatform=ARDUINO
  SPI_Config_out : arduinolib/SPI WriteRead  SPIModule=0  slaveSelectPin_=10  blockPlatform=ARDUINO
  Temp_Out_C : Outport
  Temp_Out_Valid : Outport  Port=2
  Temp_Out_Fault : Outport  Port=3
  Temp_Out_Raw : Outport  Port=4
  wires:
  MAX31865_config/1 -> SPI_Config_out/1
  RTD_Read_command/1 -> SPI Read_RTD_out/1
  Fault_Read_Command/1 -> SPI Read_Fault_out/1
  SPI Read_RTD_out/1 -> MAX31865_Temperature Conversion/1(rtdBytes)
  SPI Read_Fault_out/1 -> MAX31865_Temperature Conversion/2(faultBytes)
  MAX31865_Temperature Conversion/1(Temp_Out_C) -> Temp_Out_C/1
  MAX31865_Temperature Conversion/2(Temp_Out_Valid) -> Temp_Out_Valid/1
  MAX31865_Temperature Conversion/3(Temp_Out_Fault) -> Temp_Out_Fault/1
  MAX31865_Temperature Conversion/4(Temp_Out_Raw) -> Temp_Out_Raw/1

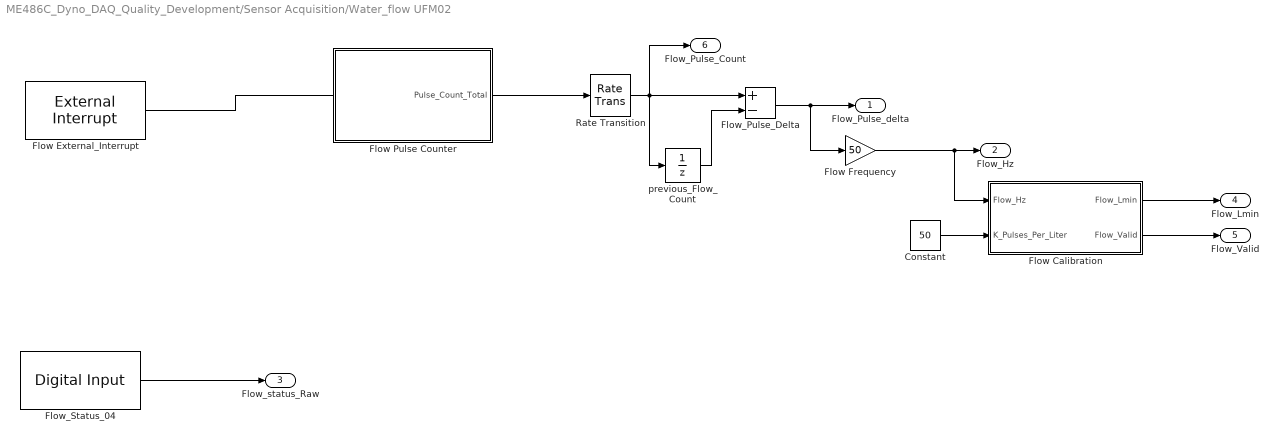
== system ME486C_Dyno_DAQ_Quality_Development/Sensor Acquisition/Water_flow UFM02 ==
  Constant : Constant  Value=50  OutDataTypeStr=double
  Flow Calibration : MATLAB Function  TreatAsAtomicUnit=on
  Flow External_Interrupt : arduinolib/External Interrupt  Pin=3  PullUp=off  Mode=RISING  InterruptSimulationInput=off
  Flow Frequency : Gain  Gain=50
  Flow Pulse Counter : Subsystem
  Flow_Pulse_Delta : Sum  Inputs=+-  AccumDataTypeStr=uint32
  Flow_Status_04 : arduinolib/Digital Input  pinNumber=4  mode=Default  Direction=input  SampleTime=0.02  blockPlatform=arduino
  Rate Transition : RateTransition
  previous_Flow_Count : UnitDelay  InitialCondition=uint32(0)  SampleTime=0.02  HasFrameUpgradeWarning=on
  Flow_Pulse_delta : Outport
  Flow_Hz : Outport  Port=2
  Flow_status_Raw : Outport  Port=3
  Flow_Lmin : Outport  Port=4
  Flow_Valid : Outport  Port=5
  Flow_Pulse_Count : Outport  Port=6
  wires:
  Flow External_Interrupt/1 -> ?
  Flow Pulse Counter/1(Pulse_Count_Total) -> Rate Transition/1
  Rate Transition/1 -> Flow_Pulse_Count/1, previous_Flow_Count/1, Flow_Pulse_Delta/1
  previous_Flow_Count/1 -> Flow_Pulse_Delta/2
  Flow_Pulse_Delta/1 -> Flow Frequency/1, Flow_Pulse_delta/1
  Flow Frequency/1 -> Flow Calibration/1(Flow_Hz), Flow_Hz/1
  Flow_Status_04/1 -> Flow_status_Raw/1
  Constant/1 -> Flow Calibration/2(K_Pulses_Per_Liter)
  Flow Calibration/1(Flow_Lmin) -> Flow_Lmin/1
  Flow Calibration/2(Flow_Valid) -> Flow_Valid/1

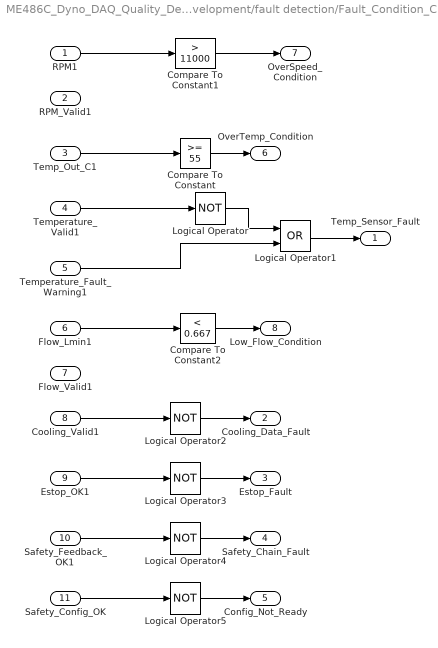
== system ME486C_Dyno_DAQ_Quality_Development/fault detection/Fault_Condition_Checks ==
  RPM1 : Inport
  RPM_Valid1 : Inport  Port=2
  Temp_Out_C1 : Inport  Port=3
  Temperature_Valid1 : Inport  Port=4
  Temperature_Fault_Warning1 : Inport  Port=5
  Flow_Lmin1 : Inport  Port=6
  Flow_Valid1 : Inport  Port=7
  Cooling_Valid1 : Inport  Port=8
  Estop_OK1 : Inport  Port=9
  Safety_Feedback_OK1 : Inport  Port=10
  Safety_Config_OK : Inport  Port=11
  Compare To Constant : simulink/Logic and Bit Operations/Compare To Constant  relop=>=  const=55  OutDataTypeStr=boolean
  Compare To Constant1 : simulink/Logic and Bit Operations/Compare To Constant  relop=>  const=11000  OutDataTypeStr=boolean
  Compare To Constant2 : simulink/Logic and Bit Operations/Compare To Constant  relop=<  const=0.667  OutDataTypeStr=boolean
  Logical Operator{,2..5} (5 alike) : Logic  Operator=NOT  AllPortsSameDT=off  OutDataTypeStr=boolean
  Logical Operator1 : Logic  Operator=OR  AllPortsSameDT=off  OutDataTypeStr=boolean
  Temp_Sensor_Fault : Outport
  Cooling_Data_Fault : Outport  Port=2
  Estop_Fault : Outport  Port=3
  Safety_Chain_Fault : Outport  Port=4
  Config_Not_Ready : Outport  Port=5
  OverTemp_Condition : Outport  Port=6
  OverSpeed_Condition : Outport  Port=7
  Low_Flow_Condition : Outport  Port=8
  wires:
  Temperature_Valid1/1 -> Logical Operator/1
  Logical Operator/1 -> Logical Operator1/1
  Temperature_Fault_Warning1/1 -> Logical Operator1/2
  Logical Operator1/1 -> Temp_Sensor_Fault/1
  Cooling_Valid1/1 -> Logical Operator2/1
  Logical Operator2/1 -> Cooling_Data_Fault/1
  Estop_OK1/1 -> Logical Operator3/1
  Logical Operator3/1 -> Estop_Fault/1
  Safety_Feedback_OK1/1 -> Logical Operator4/1
  Logical Operator4/1 -> Safety_Chain_Fault/1
  Safety_Config_OK/1 -> Logical Operator5/1
  Logical Operator5/1 -> Config_Not_Ready/1
  Temp_Out_C1/1 -> Compare To Constant/1
  Compare To Constant/1 -> OverTemp_Condition/1
  RPM1/1 -> Compare To Constant1/1
  Compare To Constant1/1 -> OverSpeed_Condition/1
  Flow_Lmin1/1 -> Compare To Constant2/1
  Compare To Constant2/1 -> Low_Flow_Condition/1

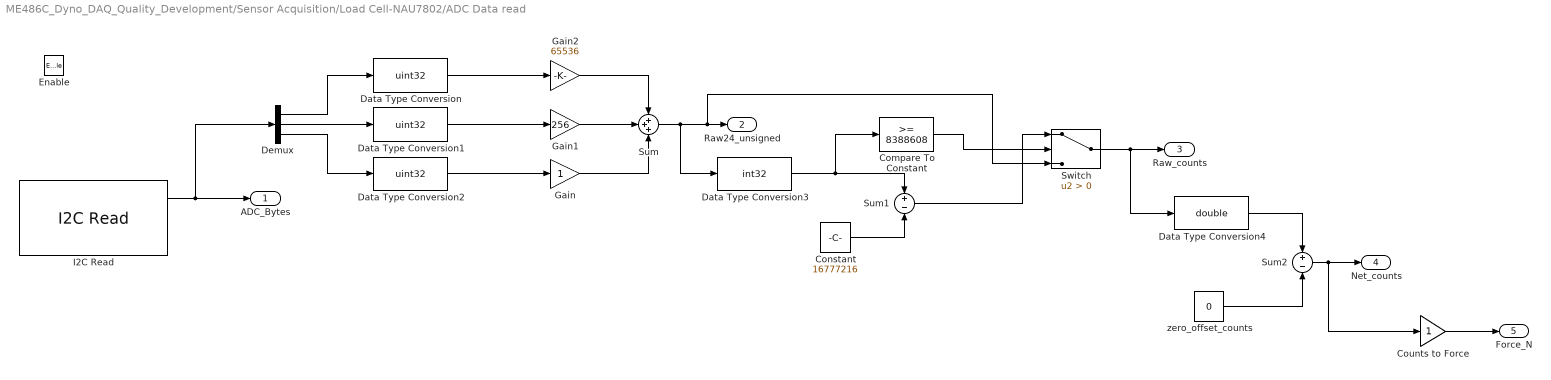
== system ME486C_Dyno_DAQ_Quality_Development/Sensor Acquisition/Load Cell-NAU7802/ADC Data read ==
  Enable : EnablePort
  Compare To Constant : simulink/Logic and Bit Operations/Compare To Constant  relop=>=  const=8388608  OutDataTypeStr=boolean
  Constant : Constant  Value=16777216
  Counts to Force : Gain
  Data Type Conversion : DataTypeConversion  OutDataTypeStr=uint32  SaturateOnIntegerOverflow=off  RndMeth=Floor
  Data Type Conversion1 : DataTypeConversion  OutDataTypeStr=uint32  SaturateOnIntegerOverflow=off  RndMeth=Floor
  Data Type Conversion2 : DataTypeConversion  OutDataTypeStr=uint32  SaturateOnIntegerOverflow=off  RndMeth=Floor
  Data Type Conversion3 : DataTypeConversion  OutDataTypeStr=int32  SaturateOnIntegerOverflow=off  RndMeth=Floor
  Data Type Conversion4 : DataTypeConversion  OutDataTypeStr=double  SaturateOnIntegerOverflow=off  RndMeth=Floor
  Demux : Demux  Outputs=3
  Gain : Gain
  Gain1 : Gain  Gain=256
  Gain2 : Gain  Gain=65536
  I2C Read : arduinolib/I2C Read  I2CModule=0  Mode=Master  SlaveAddress=hex2dec('2A')  SlaveByteOrder=BigEndian  Direction=Receiver  RegisterAddressMode=on  RegisterAddress=hex2dec('12')  SlaveDataType=uint8  DataLength=3  NoAck=off  RepeatedStart=off  OutputStatus=on  blockPlatform=ARDUINO  SampleTime=0.02
  Sum : Sum  Inputs=+++
  Sum1 : Sum  Inputs=+-
  Sum2 : Sum  Inputs=+-
  Switch : Switch  Criteria=u2 > Threshold  SaturateOnIntegerOverflow=off  InputSameDT=off
  zero_offset_counts : Constant  Value=0  OutDataTypeStr=double
  ADC_Bytes : Outport
  Raw24_unsigned : Outport  Port=2
  Raw_counts : Outport  Port=3
  Net_counts : Outport  Port=4
  Force_N : Outport  Port=5
  wires:
  I2C Read/1 -> Demux/1, ADC_Bytes/1
  Demux/1 -> Data Type Conversion/1
  Demux/2 -> Data Type Conversion1/1
  Demux/3 -> Data Type Conversion2/1
  Data Type Conversion1/1 -> Gain1/1
  Data Type Conversion2/1 -> Gain/1
  Data Type Conversion/1 -> Gain2/1
  Gain1/1 -> Sum/2
  Gain/1 -> Sum/3
  Sum/1 -> Data Type Conversion3/1, Switch/3, Raw24_unsigned/1
  Gain2/1 -> Sum/1
  Data Type Conversion3/1 -> Sum1/1, Compare To Constant/1
  Constant/1 -> Sum1/2
  Sum1/1 -> Switch/1
  Compare To Constant/1 -> Switch/2
  Switch/1 -> Data Type Conversion4/1, Raw_counts/1
  Data Type Conversion4/1 -> Sum2/1
  zero_offset_counts/1 -> Sum2/2
  Sum2/1 -> Counts to Force/1, Net_counts/1
  Counts to Force/1 -> Force_N/1

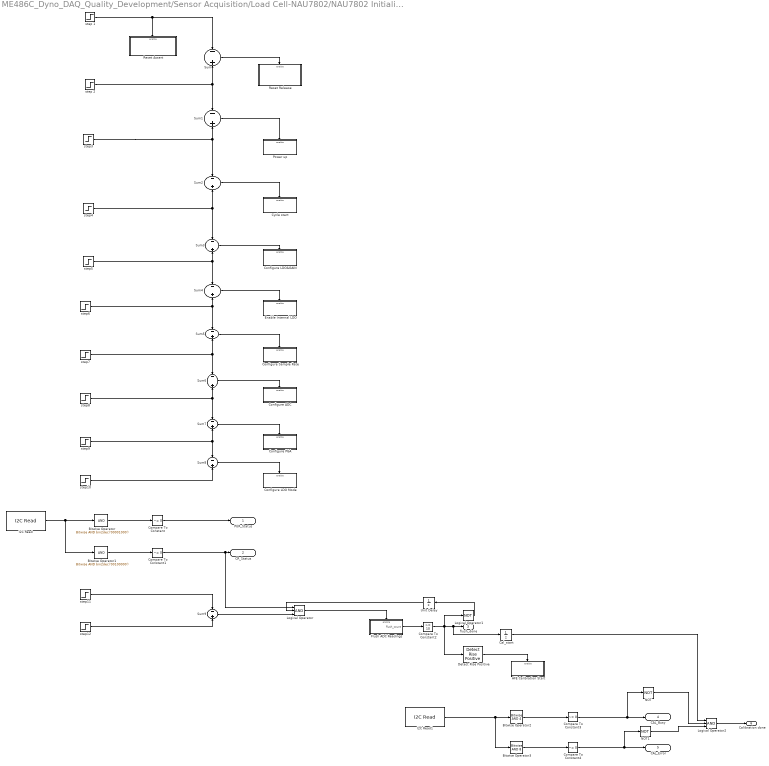
== system ME486C_Dyno_DAQ_Quality_Development/Sensor Acquisition/Load Cell-NAU7802/NAU7802 Initialization ==
  " Configure ADC" : Subsystem  TreatAsAtomicUnit=on
  AFE Calibration Start : Subsystem  TreatAsAtomicUnit=on
  Bitwise Operator : simulink/Logic and Bit Operations/Bitwise Operator  logicop=AND  UseBitMask=on  BitMask=bin2dec('00001000')  BitMaskRealWorld=Stored Integer
  Bitwise Operator1 : simulink/Logic and Bit Operations/Bitwise Operator  logicop=AND  UseBitMask=on  BitMask=bin2dec('00100000')  BitMaskRealWorld=Stored Integer
  Bitwise Operator2 : simulink/Logic and Bit Operations/Bitwise Operator  logicop=AND  UseBitMask=on  BitMask=4  BitMaskRealWorld=Stored Integer
  Bitwise Operator3 : simulink/Logic and Bit Operations/Bitwise Operator  logicop=AND  UseBitMask=on  BitMask=8  BitMaskRealWorld=Stored Integer
  Cal_start : UnitDelay  SampleTime=-1  HasFrameUpgradeWarning=on
  Compare To Constant{,1,3..4} (4 alike) : simulink/Logic and Bit Operations/Compare To Constant  relop=~=  const=0  OutDataTypeStr=boolean
  Compare To Constant2 : simulink/Logic and Bit Operations/Compare To Constant  relop=>=  const=10  OutDataTypeStr=boolean
  Configure LDO Mode : Subsystem  TreatAsAtomicUnit=on
  Configure LDO&GAIN : Subsystem  TreatAsAtomicUnit=on
  Configure PGA : Subsystem  TreatAsAtomicUnit=on
  Configure Sample Rate : Subsystem  TreatAsAtomicUnit=on
  Cycle start : Subsystem  TreatAsAtomicUnit=on
  Detect Rise Positive : simulink/Logic and Bit Operations/Detect Rise Positive  vinit=0  OutDataTypeStr=boolean
  Enable Internal LDO : Subsystem  TreatAsAtomicUnit=on
  Flush ADC Readings : Subsystem  TreatAsAtomicUnit=on
  I2C Read : arduinolib/I2C Read  I2CModule=0  Mode=Master  SlaveAddress=hex2dec('2A')  SlaveByteOrder=BigEndian  Direction=Receiver  RegisterAddressMode=on  RegisterAddress=hex2dec('00')  SlaveDataType=uint8  DataLength=1  NoAck=off  RepeatedStart=off  OutputStatus=off  blockPlatform=ARDUINO  SampleTime=0.02
  I2C Read1 : arduinolib/I2C Read  I2CModule=0  Mode=Master  SlaveAddress=hex2dec('2A')  SlaveByteOrder=BigEndian  Direction=Receiver  RegisterAddressMode=on  RegisterAddress=hex2dec('02')  SlaveDataType=uint8  DataLength=1  NoAck=off  RepeatedStart=off  OutputStatus=off  blockPlatform=ARDUINO  SampleTime=0.02
  Logical Operator : Logic  Inputs=3  AllPortsSameDT=off  OutDataTypeStr=boolean
  Logical Operator1 : Logic  Operator=NOT  AllPortsSameDT=off  OutDataTypeStr=boolean
  Logical Operator2 : Logic  Inputs=3  AllPortsSameDT=off  OutDataTypeStr=boolean
  NOT : Logic  Operator=NOT  IconShape=distinctive  AllPortsSameDT=off  OutDataTypeStr=boolean
  NOT1 : Logic  Operator=NOT  IconShape=distinctive  AllPortsSameDT=off  OutDataTypeStr=boolean
  Power up : Subsystem  TreatAsAtomicUnit=on
  Reset Assert : Subsystem  TreatAsAtomicUnit=on
  Reset Release : Subsystem
  Sum{,1..9} (10 alike) : Sum  Inputs=-+
  Unit Delay : UnitDelay  SampleTime=-1  HasFrameUpgradeWarning=on
  step 1 : Step  Time=0.02  Before=1  After=0  SampleTime=0.02
  step 2 : Step  Time=0.04  Before=1  After=0  SampleTime=0.02
  step10 : Step  Time=0.20  Before=1  After=0  SampleTime=0.02
  step11 : Step  Time=0.46  Before=1  After=0  SampleTime=0.02
  step12 : Step  Time=0.66  Before=1  After=0  SampleTime=0.02
  step3 : Step  Time=0.06  Before=1  After=0  SampleTime=0.02
  step4 : Step  Time=0.08  Before=1  After=0  SampleTime=0.02
  step5 : Step  Time=0.1  Before=1  After=0  SampleTime=0.02
  step6 : Step  Time=0.12  Before=1  After=0  SampleTime=0.02
  step7 : Step  Time=0.14  Before=1  After=0  SampleTime=0.02
  step8 : Step  Time=0.16  Before=1  After=0  SampleTime=0.02
  step9 : Step  Time=.18  Before=1  After=0  SampleTime=0.02
  PUR_Status : Outport
  CR_Status : Outport  Port=2
  flush_done : Outport  Port=3
  CAL_Busy : Outport  Port=4
  CAL_Error : Outport  Port=5
  Calibration done : Outport  Port=6
  wires:
  step 1/1 -> Reset Assert/Enable, Sum/1
  step 2/1 -> Sum/2, Sum1/1
  Sum/1 -> Reset Release/Enable
  I2C Read/1 -> Bitwise Operator1/1, Bitwise Operator/1
  Bitwise Operator/1 -> Compare To Constant/1
  Compare To Constant/1 -> PUR_Status/1
  step3/1 -> Sum1/2, Sum2/1
  step4/1 -> Sum3/1, Sum2/2
  step5/1 -> Sum4/1, Sum3/2
  step6/1 -> Sum4/2, Sum5/1
  step7/1 -> Sum5/2, Sum6/1
  Sum2/1 -> Cycle start/Enable
  Sum1/1 -> Power up/Enable
  Sum3/1 -> Configure LDO&GAIN/Enable
  Sum4/1 -> Enable Internal LDO/Enable
  Sum5/1 -> Configure Sample Rate/Enable
  step8/1 -> Sum7/1, Sum6/2
  Sum6/1 -> " Configure ADC"/Enable
  step9/1 -> Sum8/1, Sum7/2
  Sum7/1 -> Configure PGA/Enable
  step10/1 -> Sum8/2
  Sum8/1 -> Configure LDO Mode/Enable
  Compare To Constant1/1 -> Logical Operator/1, CR_Status/1
  Bitwise Operator1/1 -> Compare To Constant1/1
  step11/1 -> Sum9/1
  step12/1 -> Sum9/2
  Sum9/1 -> Logical Operator/3
  Logical Operator/1 -> Flush ADC Readings/Enable
  Flush ADC Readings/1(flush_count) -> Compare To Constant2/1
  Compare To Constant2/1 -> Detect Rise Positive/1, Logical Operator1/1, Cal_start/1, flush_done/1
  Logical Operator1/1 -> Unit Delay/1
  Detect Rise Positive/1 -> AFE Calibration Start/Enable
  I2C Read1/1 -> Bitwise Operator3/1, Bitwise Operator2/1
  Compare To Constant3/1 -> NOT/1, CAL_Busy/1
  Bitwise Operator2/1 -> Compare To Constant3/1
  Bitwise Operator3/1 -> Compare To Constant4/1
  Compare To Constant4/1 -> NOT1/1, CAL_Error/1
  NOT/1 -> Logical Operator2/2
  NOT1/1 -> Logical Operator2/3
  Cal_start/1 -> Logical Operator2/1
  Logical Operator2/1 -> Calibration done/1
  Unit Delay/1 -> Logical Operator/2

== system ME486C_Dyno_DAQ_Quality_Development/Sensor Acquisition/RPM-Hall sensor/Pulse counter ==
  RPM PERIOD Measurment : TriggerPort  TriggerType=function-call  VariantControl=(inherit)
  Constant : Constant  OutDataTypeStr=uint32
  RPM_Period measurement : MATLAB Function  TreatAsAtomicUnit=on
  Sum : Sum
  Unit Delay : UnitDelay  InitialCondition=uint32(0)  SampleTime=-1  HasFrameUpgradeWarning=on
  Pulse_Count_total : Outport
  RPM_event : Outport  Port=2
  RPM_VALID : Outport  Port=3
  wires:
  Constant/1 -> Sum/1
  Unit Delay/1 -> Sum/2
  Sum/1 -> Pulse_Count_total/1, Unit Delay/1
  RPM_Period measurement/1(RPM_Event) -> RPM_event/1
  RPM_Period measurement/2(RPM_Valid) -> RPM_VALID/1

== system ME486C_Dyno_DAQ_Quality_Development/Sensor Acquisition/Water_flow UFM02/Flow Pulse Counter ==
  Increment_Count : Sum
  One_Pulse : Constant  Value=uint32(1)  OutDataTypeStr=uint32
  Previous_Count : UnitDelay  InitialCondition=uint32(0)  SampleTime=-1  HasFrameUpgradeWarning=on
  Pulse_Count_Total : Outport
  wires:
  One_Pulse/1 -> Increment_Count/1
  Previous_Count/1 -> Increment_Count/2
  Increment_Count/1 -> Pulse_Count_Total/1, Previous_Count/1

== system ME486C_Dyno_DAQ_Quality_Development/Sensor Acquisition/Load Cell-NAU7802/NAU7802 Initialization/ Configure ADC ==
  Enable : EnablePort
  Constant : Constant  Value=hex2dec('30')
  I2C Write : arduinolib/I2C Write  I2CModule=0  Mode=Master  SlaveAddress=hex2dec('2A')  SlaveByteOrder=BigEndian  Direction=Transmitter  RegisterAddressMode=on  RegisterAddress=hex2dec('15')  SlaveDataType=uint8  DataLength=1  NoAck=off  RepeatedStart=off  OutputStatus=off  blockPlatform=ARDUINO
  wires:
  Constant/1 -> I2C Write/1

== system ME486C_Dyno_DAQ_Quality_Development/Sensor Acquisition/Load Cell-NAU7802/NAU7802 Initialization/AFE Calibration Start ==
  Enable : EnablePort
  Constant : Constant  Value=hex2dec('34')  OutDataTypeStr=uint8
  I2C Write : arduinolib/I2C Write  I2CModule=0  Mode=Master  SlaveAddress=hex2dec('2A')  SlaveByteOrder=BigEndian  Direction=Transmitter  RegisterAddressMode=on  RegisterAddress=hex2dec('02')  SlaveDataType=uint8  DataLength=1  NoAck=off  RepeatedStart=off  OutputStatus=on  blockPlatform=ARDUINO
  wires:
  Constant/1 -> I2C Write/1

== system ME486C_Dyno_DAQ_Quality_Development/Sensor Acquisition/Load Cell-NAU7802/NAU7802 Initialization/Configure LDO Mode ==
  Enable : EnablePort
  Constant : Constant  Value=0  OutDataTypeStr=uint8
  I2C Write : arduinolib/I2C Write  I2CModule=0  Mode=Master  SlaveAddress=hex2dec('2A')  SlaveByteOrder=BigEndian  Direction=Transmitter  RegisterAddressMode=on  RegisterAddress=hex2dec('1B')  SlaveDataType=uint8  DataLength=1  NoAck=off  RepeatedStart=off  OutputStatus=off  blockPlatform=ARDUINO
  wires:
  Constant/1 -> I2C Write/1

== system ME486C_Dyno_DAQ_Quality_Development/Sensor Acquisition/Load Cell-NAU7802/NAU7802 Initialization/Configure LDO&GAIN ==
  Enable : EnablePort
  Constant : Constant  Value=hex2dec('27')  OutDataTypeStr=uint8
  I2C Write : arduinolib/I2C Write  I2CModule=0  Mode=Master  SlaveAddress=hex2dec('2A')  SlaveByteOrder=BigEndian  Direction=Transmitter  RegisterAddressMode=on  RegisterAddress=hex2dec('01')  SlaveDataType=uint8  DataLength=1  NoAck=off  RepeatedStart=off  OutputStatus=on  blockPlatform=ARDUINO
  wires:
  Constant/1 -> I2C Write/1

== system ME486C_Dyno_DAQ_Quality_Development/Sensor Acquisition/Load Cell-NAU7802/NAU7802 Initialization/Configure PGA ==
  Enable : EnablePort
  Constant : Constant  Value=hex2dec('80')  OutDataTypeStr=uint8
  I2C Write : arduinolib/I2C Write  I2CModule=0  Mode=Master  SlaveAddress=hex2dec('2A')  SlaveByteOrder=BigEndian  Direction=Transmitter  RegisterAddressMode=on  RegisterAddress=hex2dec('1C')  SlaveDataType=uint8  DataLength=1  NoAck=off  RepeatedStart=off  OutputStatus=off  blockPlatform=ARDUINO
  wires:
  Constant/1 -> I2C Write/1

== system ME486C_Dyno_DAQ_Quality_Development/Sensor Acquisition/Load Cell-NAU7802/NAU7802 Initialization/Configure Sample Rate ==
  Enable : EnablePort
  Constant : Constant  Value=hex2dec('30')  OutDataTypeStr=uint8
  I2C Write : arduinolib/I2C Write  I2CModule=0  Mode=Master  SlaveAddress=hex2dec('2A')  SlaveByteOrder=BigEndian  Direction=Transmitter  RegisterAddressMode=on  RegisterAddress=hex2dec('02')  SlaveDataType=uint8  DataLength=1  NoAck=off  RepeatedStart=off  OutputStatus=on  blockPlatform=ARDUINO
  wires:
  Constant/1 -> I2C Write/1

== system ME486C_Dyno_DAQ_Quality_Development/Sensor Acquisition/Load Cell-NAU7802/NAU7802 Initialization/Cycle start ==
  Enable : EnablePort
  Constant : Constant  Value=hex2dec('16')  OutDataTypeStr=uint8
  I2C Write : arduinolib/I2C Write  I2CModule=0  Mode=Master  SlaveAddress=hex2dec('2A')  SlaveByteOrder=BigEndian  Direction=Transmitter  RegisterAddressMode=on  RegisterAddress=hex2dec('00')  SlaveDataType=uint8  DataLength=1  NoAck=off  RepeatedStart=off  OutputStatus=off  blockPlatform=ARDUINO
  wires:
  Constant/1 -> I2C Write/1

== system ME486C_Dyno_DAQ_Quality_Development/Sensor Acquisition/Load Cell-NAU7802/NAU7802 Initialization/Enable Internal LDO ==
  Enable : EnablePort
  Constant : Constant  Value=hex2dec('96')  OutDataTypeStr=uint8
  I2C Write : arduinolib/I2C Write  I2CModule=0  Mode=Master  SlaveAddress=hex2dec('2A')  SlaveByteOrder=BigEndian  Direction=Transmitter  RegisterAddressMode=on  RegisterAddress=hex2dec('00')  SlaveDataType=uint8  DataLength=1  NoAck=off  RepeatedStart=off  OutputStatus=on  blockPlatform=ARDUINO
  wires:
  Constant/1 -> I2C Write/1
